simulink model "filter_current"  (R2024b)
settings: configuration reference "MCConfiguration" (kept outside this file)
model workspace (MAT data in the model file):
  FilterCurrent_Ts : Simulink.Parameter (value not decoded)
libraries: dspstat3 x1
settings Model: DataDictionary=embeddedBoard_common.sldd  Creator=ascalzo  LastModifiedBy=mfussi
settings ConfigSetRef: SourceName=MCConfiguration

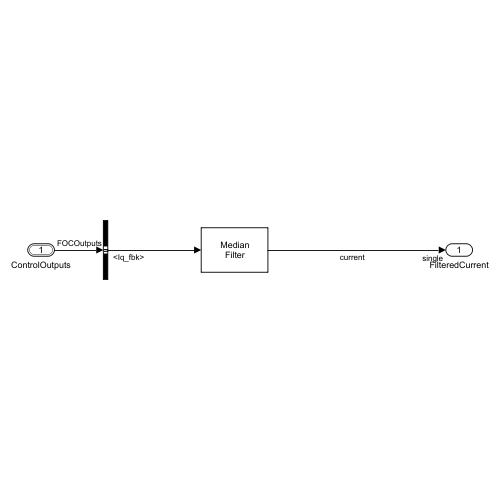
[thumbnail: Simulink's stored preview of the top-level diagram]
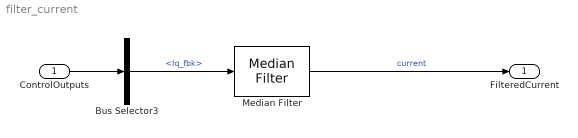
== system filter_current ==
  ControlOutputs : Inport  OutDataTypeStr=Bus: FOCOutputs  BusOutputAsStruct=on
  Bus Selector3 : BusSelector  OutputSignals=Iq_fbk
  Median Filter : dspstat3/Median Filter  WindowLength=32  SimulateUsing=Code generation
  FilteredCurrent : Outport  OutDataTypeStr=single  Unit=A  BusOutputAsStruct=on
  wires:
  ControlOutputs/1 -> Bus Selector3/1
  Bus Selector3/1 -> Median Filter/1  "<Iq_fbk>"
  Median Filter/1 -> FilteredCurrent/1  "current"
